simulink model "dc_motor_str_virtual"  (R2026a)
settings: Solver=FixedStepDiscrete  StopTime=T_exp  FixedStep=Ts
model workspace (MATLAB code in the model file):
  | % Parameters for this model (edit here, then press Ctrl+D to update)
  | Ts = 0.01;              % sample time [s]
  | T_exp = 80;             % length of the run [s] (100 s on the hardware, set below)
  | Vs = 6;                 % maximum motor voltage (motor rating, controller limit) [V]
  | V_supply = 6;           % driver supply voltage [V] (PWM duty 255 = V_supply)
  | CPR = 12*298;           % encoder counts per output-shaft revolution
  | 
  | % Speed reference: square wave between r_low and r_high
  | r_low = 20;  r_high = 40;   % [RPM]
  | r_period = 6;               % [s]
  | 
  | % Speed low-pass filter (also applied to the voltage for estimation)
  | filt_num = 0.2;  filt_den = [1 -0.8];
  | 
  | % Required closed-loop response (pole placement)
  | zeta = 1.0;             % damping ratio
  | wn = 6;                 % natural frequency [rad/s]
  | 
  | % Self-tuning PI
  | adapt_on = 1;           % 1 = self-tuning, 0 = fixed gains Kp0, Ki0
  | Kp0 = 0.1;  Ki0 = 0.5;  % gains used until the model is valid [V/RPM, V/(RPM s)]
  | Kp_max = 1;  Ki_max = 10;   % gain limits
  | 
  | % RLS estimator
  | D = 5;                  % estimate every D samples (Te = D*Ts)
  | lambda = 0.99;          % forgetting factor (0 < lambda <= 1)
  | P0 = 100;               % initial covariance, P = P0*I
  | TraceMax = 1e4;         % trace(P) limit (prevents covariance wind-up)
  | K0 = 10;  tau0 = 0.3;   % initial guess of the motor gain [RPM/V] and time constant [s]
  | 
  | % Virtual motor (illustrative values, used only by the virtual model)
  | K_true = 16;            % gain [RPM per V]
  | tau_true = 0.25;        % time constant [s]
  | V_dead = 0.5;           % dead-band (static friction) [V]
  | t_change = 40;          % time at which the motor gain changes [s]
  | K_factor = 0.6;         % new gain = K_factor*K_true (e.g. extra load)
settings Model: Creator=00782620  LastModifiedBy=00782620

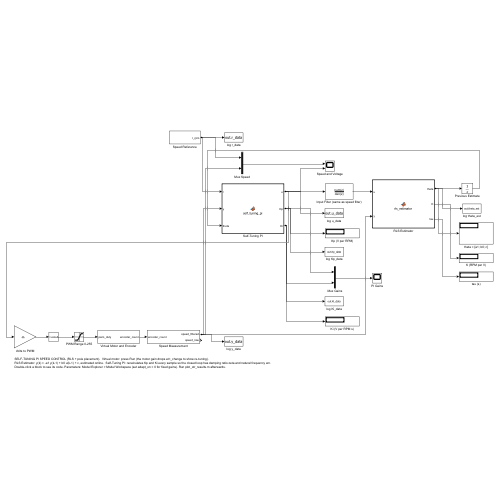
[thumbnail: Simulink's stored preview of the top-level diagram]
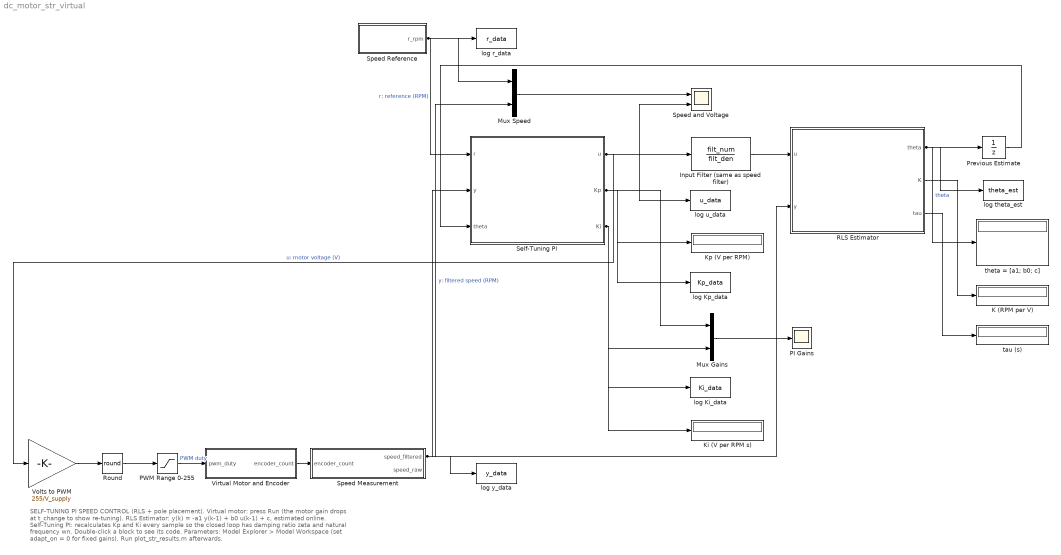
== system dc_motor_str_virtual ==
  note: SELF-TUNING PI SPEED CONTROL (RLS + pole placement).  Virtual motor: press Run (the motor gain drops at t_change to show re-tuning).
      | RLS Estimator: y(k) = -a1 y(k-1) + b0 u(k-1) + c, estimated online.  Self-Tuning PI: recalculates Kp and Ki every sample so the closed loop has damping ratio zeta and natural frequency wn.
      | Double-click a block to see its code. Parameters: Model Explorer > Model Workspace (set adapt_on = 0 for fixed gains). Run plot_str_results.m afterwards.
  Input Filter (same as speed filter) : DiscreteFilter  Numerator=filt_num  Denominator=filt_den  SampleTime=Ts
  K (RPM per V) : Display
  Ki (V per RPM s) : Display
  Kp (V per RPM) : Display
  Mux Gains : Mux  Inputs=2
  Mux Speed : Mux  Inputs=2
  PI Gains : Scope
  PWM Range 0-255 : Saturate  UpperLimit=255  LowerLimit=0
  Previous Estimate : UnitDelay  InitialCondition=[-exp(-D*Ts/tau0); K0*(1 - exp(-D*Ts/tau0)); 0]  SampleTime=Ts
  RLS Estimator : MATLAB Function  TreatAsAtomicUnit=on
  Round : Rounding  Operator=round
  Self-Tuning PI : MATLAB Function  TreatAsAtomicUnit=on
  Speed Measurement : Subsystem
  Speed Reference : Subsystem
  Speed and Voltage : Scope  NumInputPorts=2
  Virtual Motor and Encoder : Subsystem
  Volts to PWM : Gain  Gain=255/V_supply
  log Ki_data : ToWorkspace  VariableName=Ki_data  SampleTime=-1
  log Kp_data : ToWorkspace  VariableName=Kp_data  SampleTime=-1
  log r_data : ToWorkspace  VariableName=r_data  SampleTime=-1
  log theta_est : ToWorkspace  VariableName=theta_est  SampleTime=-1
  log u_data : ToWorkspace  VariableName=u_data  SampleTime=-1
  log y_data : ToWorkspace  VariableName=y_data  SampleTime=-1
  tau (s) : Display
  theta = [a1; b0; c] : Display
  wires:
  Volts to PWM/1 -> Round/1
  Round/1 -> PWM Range 0-255/1
  Speed Measurement/1(speed_filtered) -> Mux Speed/2, RLS Estimator/2(y), log y_data/1, Self-Tuning PI/2(y)  "y: filtered speed (RPM)"
  Self-Tuning PI/1(u) -> Input Filter (same as speed filter)/1, Volts to PWM/1, Speed and Voltage/2, log u_data/1  "u: motor voltage (V)"
  Virtual Motor and Encoder/1(encoder_count) -> Speed Measurement/1(encoder_count)
  PWM Range 0-255/1 -> Virtual Motor and Encoder/1(pwm_duty)  "PWM duty"
  RLS Estimator/1(theta) -> Previous Estimate/1, log theta_est/1, theta = [a1; b0; c]/1  "theta"
  Mux Speed/1 -> Speed and Voltage/1
  Speed Reference/1(r_rpm) -> Self-Tuning PI/1(r), Mux Speed/1, log r_data/1  "r: reference (RPM)"
  Self-Tuning PI/2(Kp) -> Mux Gains/1, Kp (V per RPM)/1, log Kp_data/1
  Self-Tuning PI/3(Ki) -> Ki (V per RPM s)/1, Mux Gains/2, log Ki_data/1
  Input Filter (same as speed filter)/1 -> RLS Estimator/1(u)
  Mux Gains/1 -> PI Gains/1
  RLS Estimator/2(K) -> K (RPM per V)/1
  RLS Estimator/3(tau) -> tau (s)/1
  Previous Estimate/1 -> Self-Tuning PI/3(theta)

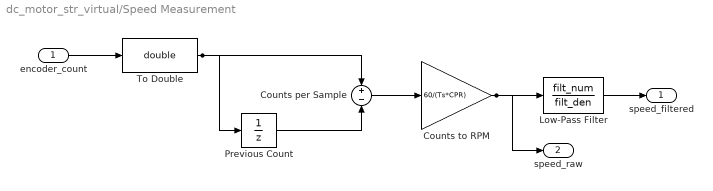
== system dc_motor_str_virtual/Speed Measurement ==
  encoder_count : Inport
  Counts per Sample : Sum  Inputs=+-
  Counts to RPM : Gain  Gain=60/(Ts*CPR)
  Low-Pass Filter : DiscreteFilter  Numerator=filt_num  Denominator=filt_den  SampleTime=Ts
  Previous Count : UnitDelay  SampleTime=Ts
  To Double : DataTypeConversion  OutDataTypeStr=double  SaturateOnIntegerOverflow=off  RndMeth=Floor
  speed_filtered : Outport
  speed_raw : Outport  Port=2
  wires:
  Counts per Sample/1 -> Counts to RPM/1
  encoder_count/1 -> To Double/1
  To Double/1 -> Counts per Sample/1, Previous Count/1
  Previous Count/1 -> Counts per Sample/2
  Counts to RPM/1 -> Low-Pass Filter/1, speed_raw/1
  Low-Pass Filter/1 -> speed_filtered/1

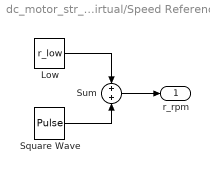
== system dc_motor_str_virtual/Speed Reference ==
  Low : Constant  Value=r_low  SampleTime=Ts
  Square Wave : DiscretePulseGenerator  Amplitude=r_high - r_low  Period=round(r_period/Ts)  PulseWidth=round(r_period/Ts/2)  PhaseDelay=round(r_period/Ts/2)  SampleTime=Ts
  Sum : Sum
  r_rpm : Outport
  wires:
  Low/1 -> Sum/1
  Square Wave/1 -> Sum/2
  Sum/1 -> r_rpm/1

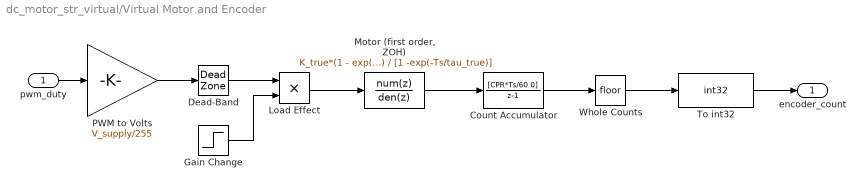
== system dc_motor_str_virtual/Virtual Motor and Encoder ==
  pwm_duty : Inport
  Count Accumulator : DiscreteTransferFcn  Numerator=[CPR*Ts/60 0]  Denominator=[1 -1]  SampleTime=Ts
  Dead-Band : DeadZone  LowerValue=-V_dead  UpperValue=V_dead
  Gain Change : Step  Time=t_change  InitialValue=1  FinalValue=K_factor  SampleTime=Ts
  Load Effect : Product
  "Motor (first order, ZOH)" : DiscreteTransferFcn  Numerator=K_true*(1 - exp(-Ts/tau_true))  Denominator=[1 -exp(-Ts/tau_true)]  SampleTime=Ts
  PWM to Volts : Gain  Gain=V_supply/255
  To int32 : DataTypeConversion  OutDataTypeStr=int32  SaturateOnIntegerOverflow=off  RndMeth=Floor
  Whole Counts : Rounding
  encoder_count : Outport
  wires:
  pwm_duty/1 -> PWM to Volts/1
  Dead-Band/1 -> Load Effect/1
  PWM to Volts/1 -> Dead-Band/1
  Gain Change/1 -> Load Effect/2
  Load Effect/1 -> "Motor (first order, ZOH)"/1
  "Motor (first order, ZOH)"/1 -> Count Accumulator/1
  Count Accumulator/1 -> Whole Counts/1
  Whole Counts/1 -> To int32/1
  To int32/1 -> encoder_count/1

== matlab function dc_motor_str_virtual/RLS Estimator ==
  data: u input; theta output; y input; K output; tau output; Ts parameter; D parameter; lambda parameter; P0 parameter; TraceMax parameter; K0 parameter; tau0 parameter
function [theta, K, tau] = rls_estimator(u, y, Ts, D, lambda, P0, TraceMax, K0, tau0)
% Recursive least squares (RLS) estimate of a first-order DC motor model
%
%   y(k) = -a1*y(k-1) + b0*u(k-1) + c,    theta = [a1; b0; c]
%   G(z) = b0/(z + a1),  K = b0/(1 + a1),  tau = -Te/ln(-a1),  Te = D*Ts
%   c is a constant term that accounts for the motor dead-band (friction).
%
%   At each estimation step:
%     phi   = [-y(k-1); u(k-1); 1]              regressor
%     e     = y(k) - phi'*theta                  prediction error
%     L     = P*phi/(lambda + phi'*P*phi)        gain vector
%     theta = theta + L*e                        update the estimate
%     P     = (P - L*phi'*P)/lambda              update the covariance
%
%   The estimate starts from an initial guess (K0, tau0). lambda < 1 lets the
%   estimate follow changes in the motor; lambda is set to 1 whenever
%   trace(P) exceeds TraceMax, to prevent covariance wind-up.
%
%   u     motor voltage [V] (passed through the same filter as the speed)
%   y     filtered motor speed [RPM]

persistent th P count uSum yPrev
if isempty(th)
    p0 = exp(-D*Ts/tau0);
    th = [-p0; K0*(1 - p0); 0];  % initial guess [a1; b0; c]
    P = P0*eye(3);             % covariance matrix
    count = D - 1;             % first estimation step at k = 0
    uSum = 0;                  % sum of u over the current interval
    yPrev = 0;                 % y at the previous estimation step
end
u = double(u);
y = double(y);

count = count + 1;
if count >= D
    uAvg = uSum/D;                       % average input over the interval
    phi = [-yPrev; uAvg; 1];             % regressor
    e = y - phi'*th;                     % prediction error
    Pphi = P*phi;
    lam = lambda;
    if trace(P) > TraceMax               % anti wind-up
        lam = 1;
    end
    L = Pphi/(lam + phi'*Pphi);          % gain vector
    th = th + L*e;                       % update the estimate
    P = (P - L*Pphi')/lam;               % update the covariance
    P = (P + P')/2;                      % keep P symmetric
    yPrev = y;
    uSum = u;                            % start the next interval
    count = 0;
else
    uSum = uSum + u;
end

theta = th;
K = 0;  tau = 0;
if abs(1 + th(1)) > 1e-9
    K = th(2)/(1 + th(1));
end
if -th(1) > 0 && -th(1) < 1
    tau = -D*Ts/log(-th(1));
end
end

== matlab function dc_motor_str_virtual/Self-Tuning PI ==
  data: r input; u output; y input; theta input; Kp output; Ki output; Ts parameter; D parameter; zeta parameter; wn parameter; Vs parameter; adapt_on parameter; Kp0 parameter; Ki0 parameter; Kp_max parameter; Ki_max parameter
function [u, Kp, Ki] = self_tuning_pi(r, y, theta, Ts, D, zeta, wn, Vs, adapt_on, Kp0, Ki0, Kp_max, Ki_max)
% Self-tuning PI speed controller (pole placement from the RLS model)
%
%   theta = [a1; b0; c] is the latest RLS model, estimated every D samples
%   (Te = D*Ts):  y(k) = -a1*y(k-1) + b0*u(k-1) + c
%
%   1. Convert the model to the control sample time Ts:
%        K = b0/(1 + a1),  p = (-a1)^(1/D),  G(z) = K*(1 - p)/(z - p)
%   2. PI controller:  C(z) = (q0*z + q1)/(z - 1),
%        q0 = Kp + Ki*Ts,  q1 = -Kp
%   3. Closed-loop characteristic equation:
%        (z - 1)(z - p) + K(1 - p)(q0*z + q1) = z^2 + p1*z + p2
%      where the required poles come from zeta and wn:
%        p1 = -2*exp(-zeta*wn*Ts)*cos(wn*Ts*sqrt(1 - zeta^2)),
%        p2 = exp(-2*zeta*wn*Ts)
%      Equating coefficients:
%        q0 = (p1 + 1 + p)/(K(1 - p)),   q1 = (p2 - p)/(K(1 - p))
%   4. Control law (velocity form, with anti-windup by clamping):
%        u(k) = u(k-1) + q0*e(k) + q1*e(k-1),   0 <= u <= Vs
%
%   The gains are only updated when the model is physically sensible
%   (0 < p < 1 and K > 0); otherwise the previous gains are kept.
%   adapt_on = 0 uses the fixed gains Kp0 and Ki0 (for comparison).

persistent uPrev ePrev KpS KiS
if isempty(uPrev)
    uPrev = 0;  ePrev = 0;  KpS = Kp0;  KiS = Ki0;
end

% ---- 1-3. recalculate the PI gains from the model ----
if adapt_on > 0
    a1 = theta(1);  b0 = theta(2);
    pe = -a1;                                % pole at the estimation rate
    if pe > 0 && pe < 1 && abs(1 + a1) > 1e-9
        K = b0/(1 + a1);                     % gain [RPM/V]
        p = pe^(1/D);                        % pole at the control rate
        if K > 0
            bs = K*(1 - p);
            if zeta < 1
                p1 = -2*exp(-zeta*wn*Ts)*cos(wn*Ts*sqrt(1 - zeta^2));
            else
                p1 = -2*exp(-zeta*wn*Ts)*cosh(wn*Ts*sqrt(zeta^2 - 1));
            end
            p2 = exp(-2*zeta*wn*Ts);
            q0 = (p1 + 1 + p)/bs;
            q1 = (p2 - p)/bs;
            KpS = min(max(-q1, 0), Kp_max);
            KiS = min(max((q0 + q1)/Ts, 0), Ki_max);
        end
    end
else
    KpS = Kp0;  KiS = Ki0;
end

% ---- 4. PI control law (velocity form) ----
e = r - double(y);
u = uPrev + (KpS + KiS*Ts)*e - KpS*ePrev;
u = min(max(u, 0), Vs);                     % actuator limits (anti-windup)
uPrev = u;
ePrev = e;
Kp = KpS;
Ki = KiS;
end
